simulink model "zad4"  (R2022b)
settings: Solver=FixedStepAuto  StartTime=0.0  StopTime=50  FixedStep=0.00001  RelTol=1e-3
model workspace (MAT data in the model file):
  a0 = 1
  a1 = 1
settings Model: Creator=vandm  LastModifiedBy=vandm

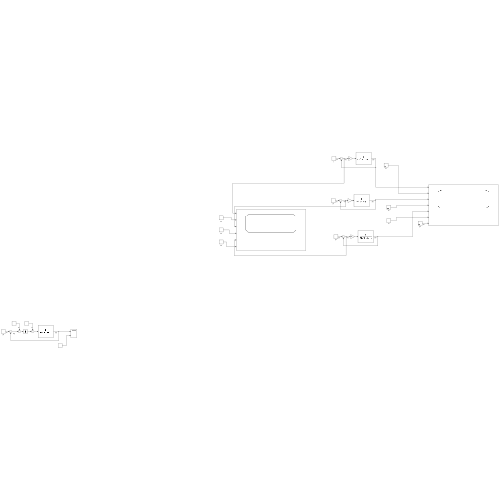
[thumbnail: Simulink's stored preview of the top-level diagram]
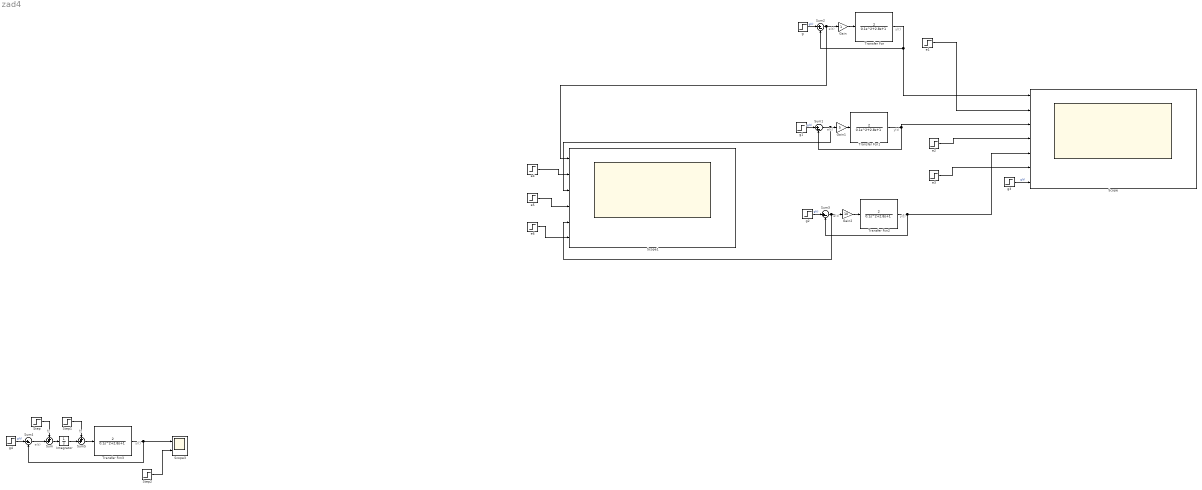
== system zad4 ==
  note: e(t)
  note: y(t)
  note: y(t)
  note: e(t)
  note: y(t)
  note: e(t)
  note: e(t)
  note: y(t)
  note: f2
  note: f1
  Gain : Gain
  Gain1 : Gain  Gain=5
  Gain2 : Gain  Gain=10
  Integrator : Integrator
  Scope : Scope  NumInputPorts=7
  Scope1 : Scope  NumInputPorts=6
  Scope3 : Scope  NumInputPorts=2
  Step : Step  Time=0  After=0  SampleTime=0
  Step1 : Step  Time=0  After=2  SampleTime=0
  Step2 : Step  Time=0  After=0  SampleTime=0
  Sum : Sum  Inputs=++|
  Sum{1..4} (4 alike) : Sum  Inputs=|+-
  Sum5 : Sum  Inputs=++|
  Transfer Fcn{,1..3} (4 alike) : TransferFcn  Numerator=[2]  Denominator=[0.1 2.8 1]
  e1 : Step  Time=0  After=3 - 3/(1 + 2)  SampleTime=0
  e2 : Step  Time=0  After=3 - 3/(1 + 2 * 5)  SampleTime=0
  e3 : Step  Time=0  After=3 - 3/(1 + 2 * 10)  SampleTime=0
  e4 : Step  Time=0  After=3/(1 + 2)  SampleTime=0
  e5 : Step  Time=0  After=3/(1 + 2 * 5)  SampleTime=0
  e6 : Step  Time=0  After=3/(1 + 2 * 10)  SampleTime=0
  g{,1..3} (4 alike) : Step  Time=0  After=3  SampleTime=0
  g4 : Step  Time=0  SampleTime=0
  wires:
  g/1 -> Sum2/1  "g(t)"
  Sum2/1 -> Scope1/1, Gain/1
  Gain/1 -> Transfer Fcn/1
  Transfer Fcn/1 -> Sum2/2, Scope/1
  e1/1 -> Scope/2
  Sum1/1 -> Scope1/3, Gain1/1
  g1/1 -> Sum1/1  "g(t)"
  Gain1/1 -> Transfer Fcn1/1
  Transfer Fcn1/1 -> Scope/3, Sum1/2
  e2/1 -> Scope/4
  Transfer Fcn2/1 -> Scope/5, Sum3/2
  g2/1 -> Sum3/1  "g(t)"
  Gain2/1 -> Transfer Fcn2/1
  Sum3/1 -> Scope1/5, Gain2/1
  e3/1 -> Scope/6
  g3/1 -> Scope/7  "g(t)"
  e4/1 -> Scope1/2
  e5/1 -> Scope1/4
  e6/1 -> Scope1/6
  Transfer Fcn3/1 -> Scope3/1, Sum4/2
  g4/1 -> Sum4/1  "g(t)"
  Sum4/1 -> Sum/2
  Step/1 -> Sum/1
  Sum/1 -> Integrator/1
  Integrator/1 -> Sum5/2
  Sum5/1 -> Transfer Fcn3/1
  Step1/1 -> Sum5/1
  Step2/1 -> Scope3/2
